simulink model "PMSM_SMO_ClosedLoop"  (R2026a)
settings: Solver=ode4  StopTime=.5  FixedStep=timing_h  MaxStep=1e-6
InitFcn:
  | pmsm_sensorless_v2_init(bdroot);
model workspace (MATLAB code in the model file + MAT data in the model file):
  T = 1e-6    (= 1e-06)
  MotorProfile = 'CHENSHA 200W / firmware profile revision 2'
  MotorSourceCommit = '48d6e86814ac6657b1313b4c92ef24c88f492e07'
  Pn = 200
  Un = 24
  Vdc = 24
  I_rated_rms = 11.5
  I_peak_rms = 23
  In = sqrt(2)*I_rated_rms
  I_peak = sqrt(2)*I_peak_rms
  n = 3000
  p = 5
  Rs = 0.105125
  Ld = 103.7615e-6    (= 0.0001037615)
  Lq = 103.7615e-6    (= 0.0001037615)
  Ls = Ld    (= 0.0001037615)
  phis = 0.06/(sqrt(2)*1.5*p)
  J = 32e-6    (= 3.2e-05)
  F = 0
  Kt = 1.5*p*phis
  Tn = 0.69
  T_peak = 1.38
  Iq_limit = 8
  accel_limit_rad_s2 = 1200
  speed_peak_rad_s = 335
  I_protection_A = 10
  Vbus_protection_high_V = 30
  Vbus_protection_low_V = 10
  RE = 10000
  rr = 2*pi/RE    (= 0.000628318530718)
  encoder_direction = -1
  fN = p*n/60    (= 250)
  wN = 2*pi*fN    (= 1570.79632679)
  ki_p = 0.8
  ki_i = 1
  fc = 20e3    (= 20000)
  Ts = 1/fc    (= 5e-05)
  dt = Ts    (= 5e-05)
  Ts_speed = 2*dt    (= 0.0001)
  w_sb = 2*pi*fN*1.2    (= 1884.95559215)
  fcb = 1000
  fwb = 50
  wc = 2*pi*fcb    (= 6283.18530718)
  wsc = 2*pi*fwb    (= 314.159265359)
  K = 30/pi    (= 9.54929658551)
  kp_w = 0.00069087230807625508    (= 0.000690872308076)
  ki_w = 0.04340878735241975    (= 0.0434087873524)
  ks_w = 0.98718608264211138    (= 0.987186082642)
  kp_id = 0.7539822368615503    (= 0.753982236862)
  ki_id = 879.64594300514204    (= 879.645943005)
  ks_id = 1.1309733552923253    (= 1.13097335529)
  kp_iq = 0.7539822368615503    (= 0.753982236862)
  ki_iq = 879.64594300514204    (= 879.645943005)
  ks_iq = 1.1309733552923253    (= 1.13097335529)
  Bm = 0
  uplimit_w = Kt*Iq_limit
  downlimit_w = -uplimit_w
  uplimit_id = Vdc/sqrt(3)
  downlimit_id = -uplimit_id
  uplimit_iq = Vdc/sqrt(3)
  downlimit_iq = -uplimit_iq
  teaching_Ts_speed = Ts_speed    (= 0.0001)
  teach_pwm_on = 0
  teach_pwm_cycles = 1
  decoupling_enabled = 1
  voltage_utilization = 0.96
  timing_on = 0
  timing_h = 1e-6    (= 1e-06)
  timing_control_sample = dt    (= 5e-05)
  timing_speed_sample = Ts_speed    (= 0.0001)
  timing_static_math = -1
  timing_carrier_y = [0 Ts/2 0]
  timing_adc_cfg = [0 0 0 1e-6 Ts 24.375e-6 1.1875e-6 1.5e-6 0 .5e-6 2]
  timing_pwm_cfg = [0 1e-6 Ts 24.375e-6 1.1875e-6 1.5e-6 0 5e-6 0 4000]
  dead_gate_on = 0
  dead_h = 1e-6    (= 1e-06)
  dead_gate_cfg = [0 1e-6 .5e-6]
  dead_comp_cfg = [0 .5e-6 Ts .05]
  dead_bridge_cfg = [p phis .01 0 .01 .7]
  sless_adc_mode = [1 0]
  sless_cfg = [0.105125 0.0001037615 5e-05 0.950604638176 0.469872645179 70 14 0.2 0.028048810878 0.777767679172 1332.66360365 888264.396098 ... (18 elements, 1x18)]
  sless_closed_cfg = [5e-05 2.8875e-05 5 0.04 0.06 0.14 1200 6 6 0.18 0.02 0.04 ... (20 elements, 1x20)]
  sless_direction = 1
  sless_enabled = 1
  sless_v2_cfg = [6.25e-08 5e-05 0.0001 2.4375e-05 1.1875e-06 1.5e-06 0 0 3e-06 5e-06 2e-06 6e-05 ... (35 elements, 1x35)]
  sless_v2_interference_s = 0
  sless_voltage_cfg = [6.25e-08 5e-05 2.8875e-05 0.105125 0.0001037615 1]
undefined symbols (not defined in the file): DiscIntNeverNeededParam
libraries: simulink x3
(part 3 of 3)

== system PMSM_SMO_ClosedLoop/无感观测/观测/角度与速度_信号3 ==
  合并 : Mux  Inputs=2
  数值1 : DataTypeConversion  OutDataTypeStr=double  SaturateOnIntegerOverflow=off  RndMeth=Floor
  数值2 : DataTypeConversion  OutDataTypeStr=double  SaturateOnIntegerOverflow=off  RndMeth=Floor
  环绕误差 : Fcn  Expr=atan2(sin(u(1)-u(2)),cos(u(1)-u(2)))*180/pi
  通道1 : Fcn  Expr=u(1)
  通道2 : Fcn  Expr=u(1)
  输出 : Outport
  wires:
  [SLessV2_theta] -> 数值1/1
  数值1/1 -> 通道1/1
  通道1/1 -> 合并/1  "估计"
  [SLessV2_truth_theta] -> 数值2/1
  数值2/1 -> 通道2/1
  通道2/1 -> 合并/2  "真值"
  合并/1 -> 环绕误差/1
  环绕误差/1 -> 输出/1

== system PMSM_SMO_ClosedLoop/无感观测/观测/角度与速度_信号4 ==
  合并 : BusCreator  Inputs=3
  数值1 : DataTypeConversion  OutDataTypeStr=double  SaturateOnIntegerOverflow=off  RndMeth=Floor
  数值2 : DataTypeConversion  OutDataTypeStr=double  SaturateOnIntegerOverflow=off  RndMeth=Floor
  数值3 : DataTypeConversion  OutDataTypeStr=double  SaturateOnIntegerOverflow=off  RndMeth=Floor
  通道1 : Fcn  Expr=u(1)*1
  通道2 : Fcn  Expr=u(1)*1
  通道3 : Fcn  Expr=u(1)*1
  输出 : Outport
  wires:
  [SLessV2_valid] -> 数值1/1
  数值1/1 -> 通道1/1
  通道1/1 -> 合并/1  "观测锁定"
  [SLessV2_state] -> 数值2/1
  数值2/1 -> 通道2/1
  通道2/1 -> 合并/2  "状态"
  [SLessV2_saturated] -> 数值3/1
  数值3/1 -> 通道3/1
  通道3/1 -> 合并/3  "饱和"
  合并/1 -> 输出/1

== matlab function PMSM_SMO_ClosedLoop/无感观测/区间电压/非理想累计 ==
  settings: updateMethod=DISCRETE  sampleTime=timing_h
  data: t input double size=1; weighted output double size=[2 1]; threshold input double size=[1 3]; carrier input double size=1; bus input double size=1; diag input double size=[1 12]; current input double size=[3 1]; vector_previous input double size=[2 1]; omega_previous input double size=1; direction input double size=1; cfg input double size=[1 35]; interval output double size=[2 1]; ready output boolean size=1; native output double size=[36 1]; uncertainty output double size=[2 1]; adc_valid input boolean size=1
function [weighted,interval,ready,native,uncertainty]=sless_direct_voltage_block(t,threshold,carrier,bus,diag,current,vector_previous,omega_previous,direction,cfg,adc_valid)
%#codegen
% Reuse the causal voltage equations; only valid ADC data can anchor them.
persistent s
if isempty(s),s=sensorless_v2_voltage_state;end
c=sensorless_v2_config_rt(cfg);
[s,weighted,interval,ready,native,uncertainty]=sensorless_r2_voltage_step(s,t,threshold,carrier,bus,diag(7),current,vector_previous,omega_previous,direction,c,adc_valid);
end

== matlab function PMSM_SMO_ClosedLoop/无感观测/执行许可/复位 ==
  settings: updateMethod=DISCRETE  sampleTime=timing_control_sample
  data: ready input boolean size=1; reset output boolean size=1; enabled input double size=1
function reset=sless_reset_block(ready,enabled)
%#codegen
reset=~ready||enabled==0;
end

== matlab function PMSM_SMO_ClosedLoop/无感观测/反电动势/滤波校正 ==
  settings: updateMethod=DISCRETE  sampleTime=timing_control_sample
  data: injection input double size=[2 1]; emf output double size=[2 1]; omega_previous input double size=1; direction input double size=1; valid input boolean size=1; reset input boolean size=1; cfg input double size=[1 18]; vector output double size=[2 1]; raw_angle output double size=1; phase output double size=1; magnitude output double size=1; front_cfg input double size=[1 35]; front_phase output double size=1
function [emf,vector,raw_angle,phase,magnitude,front_phase]=sless_v2_emf_block(injection,omega_previous,direction,valid,reset,cfg,front_cfg)
%#codegen
persistent previous
if isempty(previous),previous=zeros(2,1);end
c=sensorless_rt_config(cfg);f=sensorless_v2_config_rt(front_cfg);
if reset,omega_previous=0;end
[previous,d]=sensorless_emf_step(previous,injection,omega_previous,direction,c,valid,reset);
[front_phase,~]=sensorless_v2_front_phase(omega_previous,f);
emf=previous;rotation=[cos(front_phase) -sin(front_phase);sin(front_phase) cos(front_phase)];
vector=rotation*d.vector;raw_angle=d.raw_theta;phase=d.phase_correction;magnitude=d.magnitude;
end

== matlab function PMSM_SMO_ClosedLoop/无感观测/锁相环/归一化PLL ==
  settings: updateMethod=DISCRETE  sampleTime=timing_control_sample
  data: vector input double size=[2 1]; theta output double size=1; magnitude input double size=1; direction input double size=1; valid input boolean size=1; reset input boolean size=1; enabled input double size=1; cfg input double size=[1 18]; omega output double size=1; error output double size=1; integral output double size=1; saturated output boolean size=1; speed output double size=1
function [theta,omega,error,integral,saturated,speed]=sless_pll_block(vector,magnitude,direction,valid,reset,enabled,cfg)
%#codegen
persistent previous
if isempty(previous),previous=struct('theta',0,'integral',0,'omega',0);end
c=sensorless_rt_config(cfg);
permission=enabled~=0&&valid&&direction~=0&&magnitude>=c.validity.emf_off_below_V;
[previous,diag]=sensorless_pll_step(previous,vector,c,permission,reset);
theta=diag.theta;omega=diag.omega;error=diag.error;
integral=diag.integral;saturated=diag.saturated;speed=omega/c.pole_pairs*60/(2*pi);
end

== matlab function PMSM_SMO_ClosedLoop/无感观测/有效判断/锁定判断 ==
  settings: updateMethod=DISCRETE  sampleTime=timing_control_sample
  data: residual input double size=[2 1]; valid output boolean size=1; error input double size=1; magnitude input double size=1; saturated input boolean size=1; sample_valid input boolean size=1; direction input double size=1; reset input boolean size=1; cfg input double size=[1 18]; state output double size=1; history output double size=[3 1]
function [valid,state,history]=sless_validity_block(residual,error,magnitude,saturated,sample_valid,direction,reset,cfg)
%#codegen
persistent previous
c=sensorless_rt_config(cfg);
if isempty(previous),previous=sensorless_state(c);end
[previous,valid,state]=sensorless_validity_step(previous,residual,error,magnitude,saturated,sample_valid,direction,reset,c);
history=[previous.lock_count;previous.history_count;previous.unlock_count];
end

== matlab function PMSM_SMO_ClosedLoop/无感观测/发布许可/完成后发布 ==
  settings: updateMethod=DISCRETE  sampleTime=timing_h
  data: t input double size=1; values output double size=[13 1]; theta input double size=1; omega input double size=1; observer_valid input boolean size=1; input_valid input boolean size=1; timing_valid input boolean size=1; cfg input double size=[1 35]; permit output boolean size=1; reason output double size=1
function [values,permit,reason]=sless_direct_queue_block(t,theta,omega,observer_valid,input_valid,timing_valid,cfg)
%#codegen
% Normal JEOS capture and delayed publication, without injected events.
persistent queue integrity_latched
if isempty(queue),queue=sensorless_v2_queue_state;integrity_latched=false;end
c=sensorless_v2_config_rt(cfg);tick=round(t/c.h_s);N=round(c.period_s/c.h_s);
first=round((c.adc_trigger_s+c.adc_sync_s+3*c.adc_rank_s)/c.h_s);
new_capture=tick>=first&&mod(tick-first,N)==0&&tick~=queue.last_capture;
[queue,values,permit,reason]=sensorless_v2_queue_step(queue,t,theta,omega,observer_valid,input_valid,timing_valid,c);
if new_capture&&queue.has_pending
 queue.pending.available_time_s=(tick+ceil(c.observer_exec_s/c.h_s-1e-9))*c.h_s;
end
if bitand(uint16(reason),uint16(96))~=0,integrity_latched=true;end
if integrity_latched,permit=false;reason=double(bitor(uint16(reason),uint16(4096)));end
if ~permit,values(9:11)=0;end
end

== matlab function PMSM_SMO_ClosedLoop/无感观测/有效判断/瞬时相位许可 ==
  settings: updateMethod=DISCRETE  sampleTime=timing_control_sample
  data: theta input double size=1; packet_valid output boolean size=1; vector input double size=[2 1]; quality input boolean size=1; sample_valid input boolean size=1; reset input boolean size=1; cfg input double size=[1 18]; diagnostic output double size=[8 1]
function [packet_valid,diagnostic]=sless_r2_phase_guard_block(theta,vector,quality,sample_valid,reset,cfg)
%#codegen
[packet_valid,diagnostic]=sensorless_r2_phase_guard(theta,vector,quality,sample_valid,reset,cfg(16));
end

== matlab function PMSM_SMO_ClosedLoop/采样设置/顺序采样 ==
  settings: updateMethod=DISCRETE  sampleTime=timing_h
  data: t input; sample output size=[1 3]; current input; gates input; cfg input; diag output size=[1 15]; codes output size=[1 3]
function [sample,diag,codes] = timing_adc(t,current,gates,cfg)
%#codegen
% cfg: on, window, hold-invalid, h, Ts, trigger, aperture, rank, sync, guard, speed divider.
% Quantized event grid; outputs are published together at JEOS, in A/B/C order.
persistent captured delivered valid elapsed aperture_ok last_good raw_codes
if isempty(captured)
 captured=zeros(1,3);delivered=zeros(1,3);valid=zeros(1,3);
 elapsed=zeros(1,3);aperture_ok=ones(1,3);last_good=zeros(1,3);raw_codes=2048*ones(1,3);
end
sample=delivered;codes=raw_codes;diag=zeros(1,15);
if cfg(1)==0,return;end
h=cfg(4);N=round(cfg(5)/h);tick=round(t/h);phase=mod(tick,N);
tr=round((cfg(6)+cfg(9))/h);ap=round(cfg(7)/h);rank=round(cfg(8)/h);
guard=ceil(cfg(10)/h);pulse=zeros(1,5);
if phase==tr,pulse(1)=1;end
for k=1:3
 % Gates are sampled one grid tick earlier to avoid an algebraic gate loop.
 if gates(2*k)>0.5,elapsed(k)=elapsed(k)+1;else,elapsed(k)=0;end
 r=3-k;start=tr+r*rank;finish=start+ap;
 if phase==start,aperture_ok(k)=double(elapsed(k)>guard);end
 if phase>=start && phase<=finish && elapsed(k)<=guard,aperture_ok(k)=0;end
 if phase==finish
  valid(k)=aperture_ok(k);pulse(r+2)=1;
 end
 % Input read buffer is one tick old. Read on the following tick so the
 % captured physical value remains exactly at the aperture endpoint.
 if phase==finish+1
  captured(k)=current(k);
  % Low-side OFF has no phase-current observation. Zero is an explicit
  % teaching approximation, not a calibrated amplifier switching transient.
  if cfg(2)>0 && valid(k)==0,captured(k)=0;end
  if valid(k)>0,last_good(k)=captured(k);end
  if cfg(2)>0 && cfg(3)>0 && valid(k)==0,captured(k)=last_good(k);end
 end
end
jeos=tr+3*rank;
if phase==jeos
 delivered=captured;raw_codes=min(4095,max(0,round(2048+captured/(165/4096))));pulse(5)=1;
end
sample=delivered;codes=raw_codes;
% Phase, trigger, C/B/A hold pulses, JEOS, validity ABC, sampled ABC, sum.
diag=[phase*h pulse(1:4) pulse(5) valid delivered sum(delivered) ...
       double(mod(floor(tick/N),cfg(11))==cfg(11)-1 && phase==jeos) double(phase==jeos)];
end

== matlab function PMSM_SMO_ClosedLoop/闭环控制/启动与无感调节 ==
  settings: updateMethod=DISCRETE  sampleTime=timing_control_sample
  data: t input double size=1; theta_sample output double size=1; pub input double size=[13 1]; permit input boolean size=1; request input double size=1; cfg input double size=[1 20]; theta_pwm output double size=1; speed_feedback output double size=1; omega_feedback output double size=1; id_ref output double size=1; iq_ref output double size=1; n_ref output double size=1; state output double size=1; beta output double size=1; age output double size=1; pi_values output double size=[4 1]
function [theta_sample,theta_pwm,speed_feedback,omega_feedback,id_ref,iq_ref,n_ref,state,beta,age,pi_values]=sless_closed_control_block(t,pub,permit,request,cfg)
%#codegen
% No actual rotor angle/speed input. All state feedback is published SMO data.
persistent theta_if phase good_since switch_t integral last_iq start_id last_good theta_good omega_good speed_good
if isempty(phase)
 theta_if=0;phase=1;good_since=-1;switch_t=-1;integral=0;last_iq=0;start_id=0;
 last_good=-1;theta_good=0;omega_good=0;speed_good=0;
end
Ts=cfg(1);offset=cfg(2);pairs=cfg(3);align_end=cfg(4);rotate_s=cfg(5);ramp_end=cfg(6);
open_rpm=cfg(7);align_A=cfg(8);open_A=cfg(9);earliest=cfg(10);hold_s=cfg(11);blend_s=cfg(12);decay_s=cfg(13);
speed_ramp_s=cfg(14);Kp=cfg(15);Ki=cfg(16);Ks=cfg(17);limit=cfg(18);Kt=cfg(19);divider=round(cfg(20));
k=max(0,round((t-offset)/Ts));
open_fraction=max(0,min(1,(t-align_end)/(ramp_end-align_end)));
open_fraction=open_fraction^3*(10-15*open_fraction+6*open_fraction^2);open_speed=open_rpm*open_fraction;
open_omega=open_speed*(2*pi/60)*pairs;
if t>align_end,theta_if=mod(theta_if+Ts*open_omega,2*pi);end
if permit&&pub(1)>=0
 last_good=t;theta_good=pub(6);speed_good=pub(8);omega_good=speed_good*(2*pi/60)*pairs;
end
% Qualify the intended I/F direction and speed, using estimates only.
if permit&&pub(8)>0&&abs(pub(8)-open_speed)<=max(100,.2*open_rpm)
 if good_since<0,good_since=t;end
else,good_since=-1;
end
age=1;if last_good>=0,age=t-last_good;end
estimated=mod(theta_good+omega_good*max(0,t-last_good),2*pi);
beta=0;theta_sample=theta_if;omega_feedback=open_omega;speed_feedback=open_speed;n_ref=open_speed;
id_ref=0;iq_ref=0;
if phase==1&&t>=align_end,phase=2;end
if phase==2&&t>=earliest&&good_since>=0&&t-good_since>=hold_s-Ts/2
 phase=3;switch_t=t;
end
if phase>=3&&phase<=5&&age>1e-3,phase=6;end
if phase==1
 id_ref=align_A;
elseif phase==2
 f=max(0,min(1,(t-align_end)/rotate_s));f=f^3*(10-15*f+6*f^2);
 phi=(pi/2)*f;id_ref=align_A*cos(phi);iq_ref=open_A*sin(phi);
elseif phase==3
 beta=max(0,min(1,(t-switch_t)/blend_s));
 delta=atan2(sin(estimated-theta_if),cos(estimated-theta_if));
 theta_sample=mod(theta_if+beta*delta,2*pi);
 omega_feedback=(1-beta)*open_omega+beta*omega_good+delta/blend_s;
 speed_feedback=(1-beta)*open_speed+beta*speed_good;
 % Preserve the stator current vector while rotating the controller frame.
 id_ref=open_A*sin(beta*delta);iq_ref=open_A*cos(beta*delta);
 integral=Kt*iq_ref-Kp*(n_ref-speed_feedback);last_iq=iq_ref;
 if beta>=1,phase=4;start_id=id_ref;end
elseif phase==4||phase==5
 beta=1;theta_sample=estimated;omega_feedback=omega_good;speed_feedback=speed_good;
 closed_t=switch_t+blend_s;decay=max(0,min(1,(t-closed_t)/decay_s));id_ref=start_id*(1-decay);
 ramp=max(0,min(1,(t-closed_t-decay_s)/speed_ramp_s));n_ref=open_rpm+(request-open_rpm)*ramp;
 error=n_ref-speed_feedback;
 if mod(k,divider)==0
  raw=Kp*error+integral;torque=max(-limit,min(limit,raw));
  integral=integral+Ki*(divider*Ts)*(error-Ks*(raw-torque));last_iq=torque/Kt;
 end
 iq_ref=last_iq;
 if decay>=1,phase=5;end
else
 beta=0;id_ref=0;iq_ref=0;omega_feedback=0;speed_feedback=0;n_ref=0;
end
lead=max(0,min(Ts,pub(12)-t));theta_pwm=mod(theta_sample+omega_feedback*lead,2*pi);
proportional=Kp*(n_ref-speed_feedback);
if phase<=2,integral=Kt*iq_ref-proportional;elseif phase==6,integral=0;end
pi_values=[proportional;integral;proportional+integral;Kt*iq_ref];
state=double(phase);
end

== matlab function PMSM_SMO_ClosedLoop/SVPWM Function v1.0 ==
  data: alpha input; beta input; Vdc input; Ts input; Tcm output; sector output; diagnostic output
function [Tcm,sector,diagnostic] = fcn(alpha,beta,Vdc,Ts)
% Original six-sector construction, with simultaneous overmodulation scaling.
% Tcm is a threshold in [0,Ts/2]; upper duty = 1-2*Tcm/Ts.
% diagnostic: t1,t2,total zero-vector time,Da,Db,Dc,overmodulated,bounds_guard.
Tcm=ones(1,3)*Ts/4;sector=0;
diagnostic=[0 0 Ts .5 .5 .5 0 0];
if Vdc<=0 || Ts<=0 || (alpha==0 && beta==0),return;end
ref1=beta;ref2=(-beta+sqrt(3)*alpha)/2;ref3=(-beta-sqrt(3)*alpha)/2;
sector=4*double(ref3>0)+2*double(ref2>0)+double(ref1>0);
X=Ts*sqrt(3)/Vdc*beta;
Y=Ts*sqrt(3)/Vdc*(sqrt(3)*alpha+beta)/2;
Z=Ts*sqrt(3)/Vdc*(-sqrt(3)*alpha+beta)/2;
switch sector
 case 1,t1=Z;t2=Y;
 case 2,t1=Y;t2=-X;
 case 3,t1=-Z;t2=X;
 case 4,t1=-X;t2=Z;
 case 5,t1=X;t2=-Y;
 otherwise,t1=-Y;t2=-Z;
end
t1=max(0,t1);t2=max(0,t2);
total=t1+t2;over=double(total>Ts);
if total>Ts
 scale=Ts/total;t1=t1*scale;t2=t2*scale;
end
tzero=max(0,Ts-t1-t2);
ta=tzero/4;tb=ta+t1/2;tc=tb+t2/2;
switch sector
 case 1,Tcm=[tb ta tc];
 case 2,Tcm=[ta tc tb];
 case 3,Tcm=[ta tb tc];
 case 4,Tcm=[tc tb ta];
 case 5,Tcm=[tc ta tb];
 case 6,Tcm=[tb tc ta];
end
guard=double(any(Tcm<-1e-12) || any(Tcm>Ts/2+1e-12));
Tcm=min(Ts/2,max(0,Tcm));
diagnostic=[t1 t2 tzero 1-2*Tcm/Ts over guard];
end

== matlab function PMSM_SMO_ClosedLoop/输出延迟/CCR预装载 ==
  settings: updateMethod=DISCRETE  sampleTime=timing_h
  data: t input; applied output size=[1 3]; request input; cfg input; diag output size=[1 12]
function [applied,diag] = timing_pwm(t,request,cfg)
%#codegen
% cfg: on, h, Ts, trigger, aperture, rank, sync, compute, update mode, ARR.
% mode=0: RCR=0 update at both extrema; mode=1: underflow-only comparison.
% If a write coincides with UEV, UEV wins and the new CCR waits for the next UEV.
persistent shadow active pending shadow_seq active_seq writes stamp delay
if isempty(shadow)
 shadow=cfg(3)/4*ones(1,3);active=shadow;pending=false;
 shadow_seq=0;active_seq=0;writes=0;stamp=0;delay=0;
end
applied=active;diag=zeros(1,12);
if cfg(1)==0,return;end
h=cfg(2);N=round(cfg(3)/h);tick=round(t/h);phase=mod(tick,N);
jeos=round((cfg(4)+cfg(7)+3*cfg(6))/h);wr=jeos+round(cfg(8)/h);
update=(phase==0 || (cfg(9)==0 && phase==N/2));write=(phase==wr);
latched=false;
if update && pending
 active=shadow;active_seq=shadow_seq;pending=false;latched=true;delay=t-stamp;
end
if write
 duty=max(0,min(1,1-2*reshape(request,1,3)/cfg(3)));
 ccr=floor(duty*cfg(10)+1e-9);
 shadow=cfg(3)/2*(1-ccr/cfg(10));shadow_seq=shadow_seq+1;
 writes=writes+1;pending=true;stamp=floor(tick/N)*cfg(3)+jeos*h;
end
applied=active;
cnt=2*min(phase,N-phase)/N*cfg(10);
diag=[cnt double(phase>=N/2) double(update) double(write) double(latched) ...
 shadow_seq active_seq double(pending) delay shadow];
end

== matlab function PMSM_SMO_ClosedLoop/Universal Bridge/门极死区 ==
  settings: updateMethod=DISCRETE  sampleTime=dead_h
  data: t input; gates output size=[1 6]; request input; cfg input; blank output size=[1 3]
function [gates,blank] = gate_deadtime(t,request,cfg)
%#codegen
% cfg = [enable, event grid, programmed deadtime]. Fall immediately;
% delay each rising edge. A pulse shorter than deadtime is suppressed.
persistent previous rise armed active
if isempty(previous)
 previous=zeros(1,6);rise=zeros(1,6);armed=false(1,6);active=zeros(1,6);
end
r=double(reshape(request,1,6)>0.5);gates=r;blank=zeros(1,3);
if cfg(1)==0,return;end
assert(all(r(1:2:5)+r(2:2:6)<=1));
tick=round(t/cfg(2));delay=round(cfg(3)/cfg(2));
for k=1:6
 if r(k)==0
  active(k)=0;armed(k)=false;
 elseif previous(k)==0
  rise(k)=tick;armed(k)=true;active(k)=0;
 end
 if armed(k)&&tick-rise(k)>=delay,active(k)=1;armed(k)=false;end
end
previous=r;gates=active;
assert(all(gates(1:2:5)+gates(2:2:6)<=1));
blank=1-gates(1:2:5)-gates(2:2:6);
end

== matlab function PMSM_SMO_ClosedLoop/Universal Bridge/续流 ==
  settings: updateMethod=CONTINUOUS
  data: gates input; phase output size=[1 3]; state input; Vdc input; cfg input; diagnostic output size=[1 9]
function [phase,diagnostic] = bridge_freewheel(gates,state,Vdc,cfg)
%#codegen
% Static switched bridge for the present non-salient floating-star PMSM.
% cfg = [pole pairs, flux, zero-current band, drop enable, Ron, Vf].
% Positive current flows from pole to motor. During both-OFF, positive
% current uses the lower diode; negative current uses the upper diode.
x=reshape(state,1,4);g=reshape(gates,1,6);bus=max(Vdc,0);
theta=cfg(1)*x(4)+[0 -2*pi/3 2*pi/3];
current=x(1)*cos(theta)-x(2)*sin(theta);
emf=-cfg(1)*x(3)*cfg(2)*sin(theta);
pole=zeros(1,3);path=zeros(1,3);fixed=false(1,3);
ron=cfg(4)*cfg(5);vf=cfg(4)*cfg(6);
for k=1:3
 hi=g(2*k-1)>0.5;lo=g(2*k)>0.5;assert(~(hi&&lo));
 if hi,pole(k)=bus/2-ron*current(k);fixed(k)=true;
 elseif lo,pole(k)=-bus/2-ron*current(k);fixed(k)=true;
 elseif current(k)>cfg(3),pole(k)=-bus/2-vf;path(k)=-1;fixed(k)=true;
 elseif current(k)<-cfg(3),pole(k)=bus/2+vf;path(k)=1;fixed(k)=true;
 end
end
% Near zero, a disconnected phase follows its open-circuit EMF until a
% diode rail is reached. Small current band is a declared numerical model,
% not a device capacitance or exact diode complementarity solver.
neutral=0;
for pass=1:4
 count=sum(double(fixed));if count>0,neutral=sum((pole-emf).*double(fixed))/count;end
 changed=false;
 for k=1:3
  if ~fixed(k)
   pole(k)=emf(k)+neutral;
   if pole(k)>bus/2+vf,pole(k)=bus/2+vf;path(k)=1;fixed(k)=true;changed=true;
   elseif pole(k)<-bus/2-vf,pole(k)=-bus/2-vf;path(k)=-1;fixed(k)=true;changed=true;
   end
  end
 end
 if ~changed,break;end
end
% For near-zero open phases the neutral above enforces zero derivative;
% all fixed phases satisfy the usual floating-star mean subtraction.
phase=pole-sum(pole)/3;
diagnostic=[path pole current];
end

== matlab function PMSM_SMO_ClosedLoop/限压/死区补偿 ==
  settings: updateMethod=DISCRETE  sampleTime=timing_control_sample
  data: current input; dq output size=[1 2]; theta input; Vdc input; cfg input; diagnostic output size=[1 8]
function [dq,diagnostic] = deadtime_comp(current,theta,Vdc,cfg)
%#codegen
% cfg = [enable, compensated deadtime, PWM period, current hysteresis].
% Uses measured current ONLY. Positive phase current needs positive voltage
% correction. Correction enters BEFORE the existing final dq circle limit.
persistent polarity
if isempty(polarity),polarity=zeros(1,3);end
dq=zeros(1,2);diagnostic=zeros(1,8);
if cfg(1)==0,return;end
i=reshape(current,1,3);
for k=1:3
 if i(k)>cfg(4),polarity(k)=1;
 elseif i(k)<-cfg(4),polarity(k)=-1;
 end
end
abc=max(Vdc,0)*cfg(2)/cfg(3)*polarity;abc=abc-sum(abc)/3;
alpha=(2*abc(1)-abc(2)-abc(3))/3;beta=(abc(2)-abc(3))/sqrt(3);
dq=[alpha*cos(theta)+beta*sin(theta),-alpha*sin(theta)+beta*cos(theta)];
diagnostic=[abc dq polarity];
end

== matlab function PMSM_SMO_ClosedLoop/无感观测/采样输入/校准对齐 ==
  settings: updateMethod=DISCRETE  sampleTime=timing_control_sample
  data: t input double size=1; current output double size=[2 1]; measured input double size=[3 1]; adc input double size=[3 1]; diag input double size=[1 15]; cfg input double size=[1 35]; calibrated output double size=[3 1]; valid output boolean size=1; adc_valid output boolean size=1; timing_valid output boolean size=1; meta output double size=[12 1]
function [current,calibrated,valid,adc_valid,timing_valid,meta]=sless_v2_measure_block(t,measured,adc,diag,cfg)
%#codegen
persistent s
if isempty(s),s=sensorless_v2_measure_state;end
c=sensorless_v2_config_rt(cfg);
[s,current,calibrated,valid,adc_valid,timing_valid,meta]=sensorless_v2_measure_step(s,t,measured,adc,diag,c);
end
